simulink model "ECM_1RC_simscape_LUT"  (R2025b)
settings: Solver=ode23t  StartTime=0.0  StopTime=3500  MaxStep=0.1  RelTol=1e-3
values from neighbouring files (symbols this model uses):
  OCV_bp = [2.80555 2.85959 2.91363 3.00304 3.0606 3.09933 3.12978 3.18381 3.23096 3.26469 3.2911 3.31202 3.33368 3.35023 3.3665 3.38187 3.39652 3.40935 3.42296 3.43602 3.4475 3.45894 3.46943 3.47583 3.48131 3.48929 3.49863 3.50723 3.51419 3.52064 3.52703 3.53288 3.5383 3.54248 3.54635 3.55067 3.55538 3.56162 3.56772 3.57355 3.57907 3.58466 3.59099 3.59795 3.60491 3.61176 3.61856 3.62438 3.62996 3.63625 3.64 ...(+398 chars)    [optimiser_params_ECM_Samsung25R.m]
  SOC_bp = [0 0.01 0.02 0.03 0.04 0.05 0.06 0.07 0.08 0.09 0.1 0.11 0.12 0.13 0.14 0.15 0.16 0.17 0.18 0.19 0.2 0.21 0.22 0.23 0.24 0.25 0.26 0.27 0.28 0.29 0.3 0.31 0.32 0.33 0.34 0.35 0.36 0.37 0.38 0.39 0.4 0.41 0.42 0.43 0.44 0.45 0.46 0.47 0.48 0.49 0.5 0.51 0.52 0.53 0.54 0.55 0.56 0.57 0.58 0.59 0.6 0.61 0.62 0.63 0.64 0.65 0.66 0.67 0.68 0.69 0.7 0.71 0.72 0.73 0.74 0.75 0.76 0.77 0.78 0.79 0.8 0.81  ...(+91 chars)    [optimiser_params_ECM_Samsung25R.m]
libraries: fl_lib x9, nesl_utility x5
settings Model: Creator=klouz  LastModifiedBy=SAT

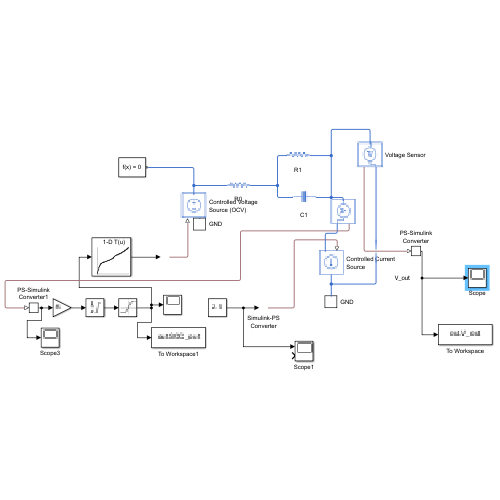
[thumbnail: Simulink's stored preview of the top-level diagram]
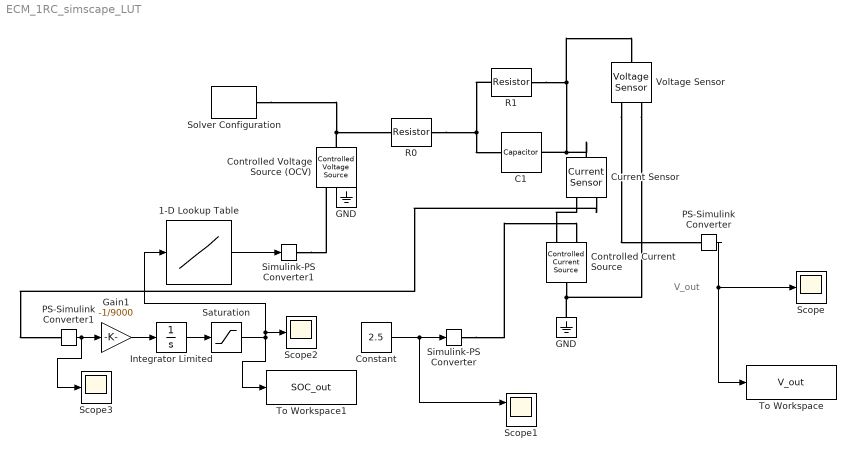
== system ECM_1RC_simscape_LUT ==
  note: V_out
  1-D Lookup Table : Lookup_n-D  NumberOfTableDimensions=1  BreakpointsForDimension1=SOC_bp  Table=OCV_bp  ExtrapMethod=Clip  InternalRulePriority=Speed  RndMeth=Simplest  LockScale=on
  C1 : fl_lib/Electrical/Electrical Elements/Capacitor  c=1000 F  r=1e-6 Ohm  g=0 1/Ohm  i_specify=off  i_priority=None  i=0 A  i_nominal_specify=off  i_nominal_value=1  i_nominal_unit=A  v_specify=off  v_priority=None  v=0 V  v_nominal_specify=off  v_nominal_value=1  v_nominal_unit=V  vc_specify=off  vc_priority=High  vc=0 V  vc_nominal_specify=off  vc_nominal_value=1  vc_nominal_unit=V
  Constant : Constant  Value=2.5
  Controlled Current Source : fl_lib/Electrical/Electrical Sources/Controlled Current Source
  "Controlled Voltage Source (OCV)  " : fl_lib/Electrical/Electrical Sources/Controlled Voltage Source
  Current Sensor : fl_lib/Electrical/Electrical Sensors/Current Sensor
  GND : fl_lib/Electrical/Electrical Elements/Electrical Reference
  "GND " : fl_lib/Electrical/Electrical Elements/Electrical Reference
  Gain1 : Gain  Gain=-1/9000
  Integrator Limited : Integrator  InitialCondition=1  LimitOutput=on  UpperSaturationLimit=1  LowerSaturationLimit=0
  PS-Simulink Converter : nesl_utility/PS-Simulink Converter  PhysicalDomain=network_engine_domain  SubClassName=ps_output  LeftPortType=input  RightPortType=output  PseudoPeriodic=off  Frequencies=[]  VectorFormat=inherit  Unit=V  AffineConversion=off
  PS-Simulink Converter1 : nesl_utility/PS-Simulink Converter  PhysicalDomain=network_engine_domain  SubClassName=ps_output  LeftPortType=input  RightPortType=output  PseudoPeriodic=off  Frequencies=[]  VectorFormat=inherit  Unit=A  AffineConversion=off
  R0 : fl_lib/Electrical/Electrical Elements/Resistor  R=0.044 Ohm  i_specify=off  i_priority=None  i=0 A  i_nominal_specify=off  i_nominal_value=1  i_nominal_unit=A  v_specify=off  v_priority=None  v=0 V  v_nominal_specify=off  v_nominal_value=1  v_nominal_unit=V
  R1 : fl_lib/Electrical/Electrical Elements/Resistor  R=0.01 Ohm  i_specify=off  i_priority=None  i=0 A  i_nominal_specify=off  i_nominal_value=1  i_nominal_unit=A  v_specify=off  v_priority=None  v=0 V  v_nominal_specify=off  v_nominal_value=1  v_nominal_unit=V
  Saturation : Saturate  UpperLimit=1  LowerLimit=0
  Scope : Scope
      settings: ActiveDisplayYMinimum=2.6517775955716512  ActiveDisplayYMaximum=4.0470016398551412
  Scope1 : Scope  NumInputPorts=2
      settings: ActiveDisplayYMinimum=-16.00955762916854  ActiveDisplayYMaximum=16.823867177928257
  Scope2 : Scope
      settings: ActiveDisplayYMinimum=-0.10404186464136778  ActiveDisplayYMaximum=1.782809771992127  DataLoggingVariableName=ScopeData2
  Scope3 : Scope
      settings: ActiveDisplayYMinimum=-0.62499999999999989  ActiveDisplayYMaximum=5.625  DataLoggingVariableName=ScopeData3
  Simulink-PS Converter : nesl_utility/Simulink-PS Converter  PhysicalDomain=network_engine_domain  SubClassName=ps_input  LeftPortType=input  RightPortType=output  PseudoPeriodic=off  Frequencies=[]  NoiseDistribution=none  NoiseParameters=[]  Unit=1  AffineConversion=off  FilteringAndDerivatives=provide  SimscapeFilterOrder=1  InputFilterTimeConstant=0.001  UdotUserProvided=0
  Simulink-PS Converter1 : nesl_utility/Simulink-PS Converter  PhysicalDomain=network_engine_domain  SubClassName=ps_input  LeftPortType=input  RightPortType=output  PseudoPeriodic=off  Frequencies=[]  NoiseDistribution=none  NoiseParameters=[]  Unit=1  AffineConversion=off  FilteringAndDerivatives=provide  SimscapeFilterOrder=1  InputFilterTimeConstant=0.001  UdotUserProvided=0
  Solver Configuration : nesl_utility/Solver Configuration  PhysicalDomain=network_engine_domain  SubClassName=solver  LeftPortType=input  RightPortType=generic  Tones=[]  Harmonics=[]  SimulateNoise=off  Profile=off  UseLocalSampling=off  EnableSwitchedLinearOptims=on  FrequencyDomain=off  UseCCode=off  RelTol=0.001  AbsTol=0.001  MinStep=1e-09  ToWorkspace=off  RevertToSquareIcSolve=off  NumHomotopyIterations=100  PhasorMode=off  PhasorModeNumHarmonics=1  ConsistencySolver=NEWTON_XTOL_AFTER_FTOL  IndexReductionMethod=DerivativeReplacement  DoDC=off  ResidualTolerance=1e-09  ConsistencyTolSource=GLOBAL  ConsistencyAbsTol=0.001  ConsistencyRelTol=0.001  ConsistencyTolFactor=0.001  UseLocalSolver=off  LocalSolverChoice=NE_BACKWARD_EULER_ADVANCER  ResolveIndetEquations=on  FunctionEvalNumThread=1  LocalSolverSampleTime=0.001  DoFixedCost=off  MaxNonlinIter=3  MaxModeIter=2  ComputeImpulses=off  ImpulseIterations=2  LinearAlgebra=auto  LinearAlgebraNumThread=0  EquationFormulation=NE_TIME_EF  DelaysMemoryBudget=1024  AutomaticFiltering=on  FilteringTimeConstant=0.001  PartitionStorageMethod=AS_NEEDED  PartitionMemoryBudget=1024  PartitionMethod=ROBUST  MultibodyUseLocalSolver=off  MultibodyLocalSolverChoice=ODE1  MultibodyLocalSolverSampleTime=0.001
  To Workspace : ToWorkspace  VariableName=V_out  SaveFormat=Timeseries  SampleTime=-1
  To Workspace1 : ToWorkspace  VariableName=SOC_out  SaveFormat=Timeseries  SampleTime=-1
  Voltage Sensor : fl_lib/Electrical/Electrical Sensors/Voltage Sensor
  wires:
  Constant/1 -> Scope1/1, Simulink-PS Converter/1
  PS-Simulink Converter/1 -> To Workspace/1, Scope/1
  Gain1/1 -> Integrator Limited/1
  Integrator Limited/1 -> Saturation/1
  1-D Lookup Table/1 -> Simulink-PS Converter1/1
  Saturation/1 -> 1-D Lookup Table/1, Scope2/1, To Workspace1/1
  PS-Simulink Converter1/1 -> Scope3/1, Gain1/1
  connections:
  R1/LConn1 -- R0/RConn1 -- C1/LConn1
  R1/RConn1 -- Voltage Sensor/LConn1 -- Current Sensor/LConn1 -- C1/RConn1
  GND/LConn1 -- "Controlled Voltage Source (OCV)  "/RConn2
  "Controlled Voltage Source (OCV)  "/LConn1 -- Solver Configuration/RConn1 -- R0/LConn1
  "GND "/LConn1 -- Controlled Current Source/LConn1 -- Voltage Sensor/RConn2
  Simulink-PS Converter/RConn1 -- Controlled Current Source/RConn1
  Voltage Sensor/RConn1 -- PS-Simulink Converter/LConn1
  Current Sensor/RConn2 -- Controlled Current Source/RConn2
  Simulink-PS Converter1/RConn1 -- "Controlled Voltage Source (OCV)  "/RConn1
  Current Sensor/RConn1 -- PS-Simulink Converter1/LConn1
